simulink model "microduck_nonlinear_state_feedback"  (R2026b)
settings: Solver=ode15s  StopTime=r.test.duration  MaxStep=r.p.cfg.sim.maxStep  RelTol=r.p.cfg.sim.relTol  AbsTol=r.p.cfg.sim.absTol
PreLoadFcn:
  | root=fileparts(get_param(bdroot,'FileName')); addpath(root,fullfile(root,'helpers')); md_expanded_cache;
PostLoadFcn:
  | md_sf_apply(bdroot);
InitFcn:
  | md_sf_apply(bdroot);
model workspace (MAT data in the model file):
  G11 = [-0.6  0; 0  -0.6]
  G12 = -12
  G13 = -4000
  G14 = [-0.6  0; 0  -0.6]
  G15 = -12
  G16 = -4000
  G17 = [-0.6  0; 0  -0.6]
  G18 = -12
  G19 = -4000
  G20 = [-0.6  0; 0  -0.6]
  G21 = -12
  G22 = -4000
  G23 = [-0.6  0; 0  -0.6]
  G24 = -12
  G25 = -4000
  G26 = [-0.6  0; 0  -0.6]
  G27 = -12
  G28 = -4000
  G29 = [-0.6  0; 0  -0.6]
  G30 = -12
  G31 = -4000
  G32 = [-0.6  0; 0  -0.6]
  G33 = -12
  G34 = -4000
  G35 = [0 0 0 0 0 0 1 0 0 0 0 0 ... (112 elements, 14x8)]
  G36 = [0 0 0 0 0 0 0.053 0 0 0 0 0 ... (112 elements, 14x8)]
  G39 = [33.3333333333 0 0 0 0 0 0 0 0 33.3333333333 0 0 ... (64 elements, 8x8)]
  G40 = [0 0 0 0 0 0 0 0 0 0 0 0 ... (112 elements, 8x14)]
  G41 = [0 0 0 0 0 0 0 0 0 0 0 0 ... (112 elements, 8x14)]
  Kd_servo = [0 0 0 0 0 0 0 0 0 0 0 0 ... (64 elements, 8x8)]
  Kp_servo = [0.55 0 0 0 0 0 0 0 0 0.55 0 0 ... (64 elements, 8x8)]
  c10 = 0
  c11 = 0
  c13 = 0
  c14 = 0
  c16 = 0
  c17 = 0
  c19 = 0
  c20 = 0
  c22 = 0
  c23 = 0
  c25 = 0
  c26 = 0
  c4 = 0
  c5 = 0
  c7 = 0
  c8 = 0
  g_world = [0; 0; -9.81]
  push_wrench = [1; 0; 0; 0; 0; 0]
  r : object (value not decoded)
  v_s2 = 2.5e-05
symbols that are objects in the model workspace (value not decoded): r
(part 2 of 5)

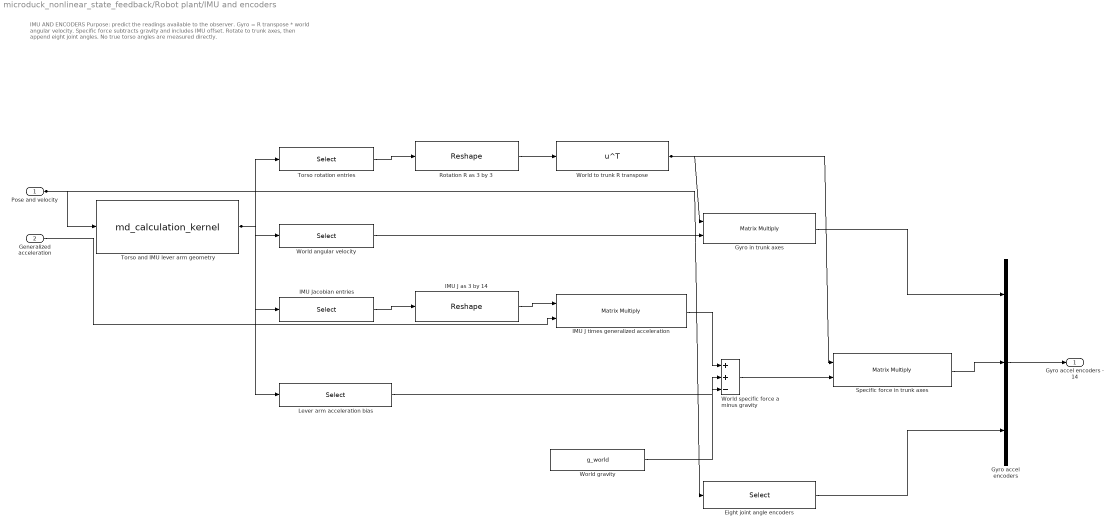
== system microduck_nonlinear_state_feedback/Robot plant/IMU and encoders ==
  note: IMU AND ENCODERS
      |
      | Purpose: predict the readings available to the observer.
      | Gyro = R transpose * world angular velocity. Specific force subtracts gravity and includes IMU offset.
      | Rotate to trunk axes, then append eight joint angles. No true torso angles are measured directly.
  Pose and velocity : Inport  Description=|
      | Pose and velocity
      | 
      | WHAT THIS BLOCK DOES
      | Receives this named signal from the parent folder. Check the name for its meaning and units.
      | 
      | FOLDER CONTEXT
      | IMU AND ENCODERS
      | 
      | Purpose: predict the readings available to the observer.
      | Gyro = R transpose * world angular velocity. Specific force subtracts gravity and includes IMU offset.
      | Rotate to trunk axes, then append eight joint angles. No true torso angles are measured directly.
  Generalized acceleration : Inport  Description=|  Port=2
      | Generalized acceleration
      | 
      | WHAT THIS BLOCK DOES
      | Receives this named signal from the parent folder. Check the name for its meaning and units.
      | 
      | FOLDER CONTEXT
      | IMU AND ENCODERS
      | 
      | Purpose: predict the readings available to the observer.
      | Gyro = R transpose * world angular velocity. Specific force subtracts gravity and includes IMU offset.
      | Rotate to trunk axes, then append eight joint angles. No true torso angles are measured directly.
  Eight joint angle encoders : Selector  Description=|  InputPortWidth=28  IndexOptions=Index vector (dialog)  Indices=[7 8 9 10 11 12 13 14]  OutputSizes=1
      | Eight joint angle encoders
      | 
      | WHAT THIS BLOCK DOES
      | Selects the labelled coordinates from an input vector without changing their physical values. Open the block to see the one-based index list.
      | 
      | FOLDER CONTEXT
      | IMU AND ENCODERS
      | 
      | Purpose: predict the readings available to the observer.
      | Gyro = R transpose * world angular velocity. Specific force subtracts gravity and includes IMU offset.
      | Rotate to trunk axes, then append eight joint angles. No true torso angles are measured directly.
  Gyro accel encoders : Mux  Description=|  Inputs=3
      | Gyro accel encoders
      | 
      | WHAT THIS BLOCK DOES
      | Joins the input vectors in port order, top to bottom. This packages signals; it does not add forces or mix units.
      | 
      | FOLDER CONTEXT
      | IMU AND ENCODERS
      | 
      | Purpose: predict the readings available to the observer.
      | Gyro = R transpose * world angular velocity. Specific force subtracts gravity and includes IMU offset.
      | Rotate to trunk axes, then append eight joint angles. No true torso angles are measured directly.
  Gyro in trunk axes : Product  Description=|  Inputs=**  Multiplication=Matrix(*)
      | Gyro in trunk axes
      | 
      | WHAT THIS BLOCK DOES
      | Multiplies/divides the inputs according to the block settings. Input operations: **. The matrix/vector dimensions must agree.
      | 
      | FOLDER CONTEXT
      | IMU AND ENCODERS
      | 
      | Purpose: predict the readings available to the observer.
      | Gyro = R transpose * world angular velocity. Specific force subtracts gravity and includes IMU offset.
      | Rotate to trunk axes, then append eight joint angles. No true torso angles are measured directly.
  IMU J as 3 by 14 : Reshape  Description=|  OutputDimensionality=Customize  OutputDimensions=[3 14]
      | IMU J as 3 by 14
      | 
      | WHAT THIS BLOCK DOES
      | Changes the arrangement of the entries into the labelled matrix shape. Entries retain MATLAB column-major order and their values do not change.
      | 
      | FOLDER CONTEXT
      | IMU AND ENCODERS
      | 
      | Purpose: predict the readings available to the observer.
      | Gyro = R transpose * world angular velocity. Specific force subtracts gravity and includes IMU offset.
      | Rotate to trunk axes, then append eight joint angles. No true torso angles are measured directly.
  IMU J times generalized acceleration : Product  Description=|  Inputs=**  Multiplication=Matrix(*)
      | IMU J times generalized acceleration
      | 
      | WHAT THIS BLOCK DOES
      | Multiplies/divides the inputs according to the block settings. Input operations: **. The matrix/vector dimensions must agree.
      | 
      | FOLDER CONTEXT
      | IMU AND ENCODERS
      | 
      | Purpose: predict the readings available to the observer.
      | Gyro = R transpose * world angular velocity. Specific force subtracts gravity and includes IMU offset.
      | Rotate to trunk axes, then append eight joint angles. No true torso angles are measured directly.
  IMU Jacobian entries : Selector  Description=|  InputPortWidth=57  IndexOptions=Index vector (dialog)  Indices=[13 14 15 16 17 18 19 20 21 22 23 24 25 26 27 28 29 30 31 32 33 34 35 36 37 38 39 40 41 42 43 44 45 46 47 48 49 50 51 52 53 54]  OutputSizes=1
      | IMU Jacobian entries
      | 
      | WHAT THIS BLOCK DOES
      | Selects the labelled coordinates from an input vector without changing their physical values. Open the block to see the one-based index list.
      | 
      | FOLDER CONTEXT
      | IMU AND ENCODERS
      | 
      | Purpose: predict the readings available to the observer.
      | Gyro = R transpose * world angular velocity. Specific force subtracts gravity and includes IMU offset.
      | Rotate to trunk axes, then append eight joint angles. No true torso angles are measured directly.
  Lever arm acceleration bias : Selector  Description=|  InputPortWidth=57  IndexOptions=Index vector (dialog)  Indices=[55 56 57]  OutputSizes=1
      | Lever arm acceleration bias
      | 
      | WHAT THIS BLOCK DOES
      | Selects the labelled coordinates from an input vector without changing their physical values. Open the block to see the one-based index list.
      | 
      | FOLDER CONTEXT
      | IMU AND ENCODERS
      | 
      | Purpose: predict the readings available to the observer.
      | Gyro = R transpose * world angular velocity. Specific force subtracts gravity and includes IMU offset.
      | Rotate to trunk axes, then append eight joint angles. No true torso angles are measured directly.
  Rotation R as 3 by 3 : Reshape  Description=|  OutputDimensionality=Customize  OutputDimensions=[3 3]
      | Rotation R as 3 by 3
      | 
      | WHAT THIS BLOCK DOES
      | Changes the arrangement of the entries into the labelled matrix shape. Entries retain MATLAB column-major order and their values do not change.
      | 
      | FOLDER CONTEXT
      | IMU AND ENCODERS
      | 
      | Purpose: predict the readings available to the observer.
      | Gyro = R transpose * world angular velocity. Specific force subtracts gravity and includes IMU offset.
      | Rotate to trunk axes, then append eight joint angles. No true torso angles are measured directly.
  Specific force in trunk axes : Product  Description=|  Inputs=**  Multiplication=Matrix(*)
      | Specific force in trunk axes
      | 
      | WHAT THIS BLOCK DOES
      | Multiplies/divides the inputs according to the block settings. Input operations: **. The matrix/vector dimensions must agree.
      | 
      | FOLDER CONTEXT
      | IMU AND ENCODERS
      | 
      | Purpose: predict the readings available to the observer.
      | Gyro = R transpose * world angular velocity. Specific force subtracts gravity and includes IMU offset.
      | Rotate to trunk axes, then append eight joint angles. No true torso angles are measured directly.
  Torso and IMU lever arm geometry : M-S-Function  Description=|  FunctionName=md_calculation_kernel  Parameters=r.p, 'imu_geometry'
      | Torso and IMU lever arm geometry
      | 
      | WHAT THIS BLOCK DOES
      | Performs the mathematical operation named on this block. Open its parameter dialog to inspect the operator and dimensions.
      | 
      | FOLDER CONTEXT
      | IMU AND ENCODERS
      | 
      | Purpose: predict the readings available to the observer.
      | Gyro = R transpose * world angular velocity. Specific force subtracts gravity and includes IMU offset.
      | Rotate to trunk axes, then append eight joint angles. No true torso angles are measured directly.
      settings: OpenFcn=edit md_rigid_body_math; edit md_calculation_kernel;
  Torso rotation entries : Selector  Description=|  InputPortWidth=57  IndexOptions=Index vector (dialog)  Indices=[1 2 3 4 5 6 7 8 9]  OutputSizes=1
      | Torso rotation entries
      | 
      | WHAT THIS BLOCK DOES
      | Selects the labelled coordinates from an input vector without changing their physical values. Open the block to see the one-based index list.
      | 
      | FOLDER CONTEXT
      | IMU AND ENCODERS
      | 
      | Purpose: predict the readings available to the observer.
      | Gyro = R transpose * world angular velocity. Specific force subtracts gravity and includes IMU offset.
      | Rotate to trunk axes, then append eight joint angles. No true torso angles are measured directly.
  World angular velocity : Selector  Description=|  InputPortWidth=57  IndexOptions=Index vector (dialog)  Indices=[10 11 12]  OutputSizes=1
      | World angular velocity
      | 
      | WHAT THIS BLOCK DOES
      | Selects the labelled coordinates from an input vector without changing their physical values. Open the block to see the one-based index list.
      | 
      | FOLDER CONTEXT
      | IMU AND ENCODERS
      | 
      | Purpose: predict the readings available to the observer.
      | Gyro = R transpose * world angular velocity. Specific force subtracts gravity and includes IMU offset.
      | Rotate to trunk axes, then append eight joint angles. No true torso angles are measured directly.
  World gravity : Constant  Description=|  Value=g_world
      | SHARED PARAMETER: g_world = r.p.g
      | Edit sf_parameters.m; per-model edits are refreshed on Run.
      | 
      | WHAT THIS BLOCK DOES
      | World gravity
      | 
      | PARAMETER
      | g_world = r.p.g
      | 
      | The short symbol is stored in this model workspace. Its numeric value is unchanged from the validated model.
  World specific force a minus gravity : Sum  Description=|  Inputs=++-
      | World specific force a minus gravity
      | 
      | WHAT THIS BLOCK DOES
      | Combines its inputs using the plus/minus signs shown on the icon. Signs: ++-.
      | 
      | FOLDER CONTEXT
      | IMU AND ENCODERS
      | 
      | Purpose: predict the readings available to the observer.
      | Gyro = R transpose * world angular velocity. Specific force subtracts gravity and includes IMU offset.
      | Rotate to trunk axes, then append eight joint angles. No true torso angles are measured directly.
  World to trunk R transpose : Math  Description=|  Operator=transpose
      | World to trunk R transpose
      | 
      | WHAT THIS BLOCK DOES
      | Performs the mathematical operation named on this block. Open its parameter dialog to inspect the operator and dimensions.
      | 
      | FOLDER CONTEXT
      | IMU AND ENCODERS
      | 
      | Purpose: predict the readings available to the observer.
      | Gyro = R transpose * world angular velocity. Specific force subtracts gravity and includes IMU offset.
      | Rotate to trunk axes, then append eight joint angles. No true torso angles are measured directly.
  Gyro accel encoders - 14 : Outport  Description=|
      | Gyro accel encoders - 14
      | 
      | WHAT THIS BLOCK DOES
      | Carries this named result out of the folder. The port number defines the interface order.
      | 
      | FOLDER CONTEXT
      | IMU AND ENCODERS
      | 
      | Purpose: predict the readings available to the observer.
      | Gyro = R transpose * world angular velocity. Specific force subtracts gravity and includes IMU offset.
      | Rotate to trunk axes, then append eight joint angles. No true torso angles are measured directly.
  wires:
  Pose and velocity/1 -> Eight joint angle encoders/1, Torso and IMU lever arm geometry/1
  Gyro in trunk axes/1 -> Gyro accel encoders/1
  Specific force in trunk axes/1 -> Gyro accel encoders/2
  Eight joint angle encoders/1 -> Gyro accel encoders/3
  World to trunk R transpose/1 -> Gyro in trunk axes/1, Specific force in trunk axes/1
  World angular velocity/1 -> Gyro in trunk axes/2
  IMU Jacobian entries/1 -> IMU J as 3 by 14/1
  IMU J as 3 by 14/1 -> IMU J times generalized acceleration/1
  Generalized acceleration/1 -> IMU J times generalized acceleration/2
  Torso and IMU lever arm geometry/1 -> IMU Jacobian entries/1, Lever arm acceleration bias/1, Torso rotation entries/1, World angular velocity/1
  Torso rotation entries/1 -> Rotation R as 3 by 3/1
  World specific force a minus gravity/1 -> Specific force in trunk axes/2
  IMU J times generalized acceleration/1 -> World specific force a minus gravity/1
  Lever arm acceleration bias/1 -> World specific force a minus gravity/2
  World gravity/1 -> World specific force a minus gravity/3
  Rotation R as 3 by 3/1 -> World to trunk R transpose/1
  Gyro accel encoders/1 -> Gyro accel encoders - 14/1

== system microduck_nonlinear_state_feedback/Robot plant/Integrate body motion ==
  note: INTEGRATE BODY MOTION
      |
      | Purpose: convert generalized acceleration into the robot pose over time.
      | First integrator: acceleration -> velocity v. Second integrator: velocity -> coordinates q.
      | The initial pose is the trimmed standing equilibrium. q and v each contain 14 values.
  In1 : Inport  Description=|
      | In1
      | 
      | WHAT THIS BLOCK DOES
      | Receives this named signal from the parent folder. Check the name for its meaning and units.
      | 
      | FOLDER CONTEXT
      | INTEGRATE BODY MOTION
      | 
      | Purpose: convert generalized acceleration into the robot pose over time.
      | First integrator: acceleration -> velocity v. Second integrator: velocity -> coordinates q.
      | The initial pose is the trimmed standing equilibrium. q and v each contain 14 values.
  Generalized velocities v : Integrator  Description=|  InitialCondition=zeros(14,1)
      | Generalized velocities v
      | 
      | WHAT THIS BLOCK DOES
      | Continuous state memory: integrates the input over time. Starts at InitialCondition = zeros(14,1).
      | 
      | FOLDER CONTEXT
      | INTEGRATE BODY MOTION
      | 
      | Purpose: convert generalized acceleration into the robot pose over time.
      | First integrator: acceleration -> velocity v. Second integrator: velocity -> coordinates q.
      | The initial pose is the trimmed standing equilibrium. q and v each contain 14 values.
  Joint and body coordinates q : Integrator  Description=|  InitialCondition=r.p.xeq(1:14)
      | Joint and body coordinates q
      | 
      | WHAT THIS BLOCK DOES
      | Continuous state memory: integrates the input over time. Starts at InitialCondition = r.p.xeq(1:14).
      | 
      | FOLDER CONTEXT
      | INTEGRATE BODY MOTION
      | 
      | Purpose: convert generalized acceleration into the robot pose over time.
      | First integrator: acceleration -> velocity v. Second integrator: velocity -> coordinates q.
      | The initial pose is the trimmed standing equilibrium. q and v each contain 14 values.
  q and v : Mux  Description=|  Inputs=2
      | q and v
      | 
      | WHAT THIS BLOCK DOES
      | Joins the input vectors in port order, top to bottom. This packages signals; it does not add forces or mix units.
      | 
      | FOLDER CONTEXT
      | INTEGRATE BODY MOTION
      | 
      | Purpose: convert generalized acceleration into the robot pose over time.
      | First integrator: acceleration -> velocity v. Second integrator: velocity -> coordinates q.
      | The initial pose is the trimmed standing equilibrium. q and v each contain 14 values.
  Out1 : Outport  Description=|
      | Out1
      | 
      | WHAT THIS BLOCK DOES
      | Carries this named result out of the folder. The port number defines the interface order.
      | 
      | FOLDER CONTEXT
      | INTEGRATE BODY MOTION
      | 
      | Purpose: convert generalized acceleration into the robot pose over time.
      | First integrator: acceleration -> velocity v. Second integrator: velocity -> coordinates q.
      | The initial pose is the trimmed standing equilibrium. q and v each contain 14 values.
  Out2 : Outport  Description=|  Port=2
      | Out2
      | 
      | WHAT THIS BLOCK DOES
      | Carries this named result out of the folder. The port number defines the interface order.
      | 
      | FOLDER CONTEXT
      | INTEGRATE BODY MOTION
      | 
      | Purpose: convert generalized acceleration into the robot pose over time.
      | First integrator: acceleration -> velocity v. Second integrator: velocity -> coordinates q.
      | The initial pose is the trimmed standing equilibrium. q and v each contain 14 values.
  Out3 : Outport  Description=|  Port=3
      | Out3
      | 
      | WHAT THIS BLOCK DOES
      | Carries this named result out of the folder. The port number defines the interface order.
      | 
      | FOLDER CONTEXT
      | INTEGRATE BODY MOTION
      | 
      | Purpose: convert generalized acceleration into the robot pose over time.
      | First integrator: acceleration -> velocity v. Second integrator: velocity -> coordinates q.
      | The initial pose is the trimmed standing equilibrium. q and v each contain 14 values.
  wires:
  In1/1 -> Generalized velocities v/1
  Generalized velocities v/1 -> Joint and body coordinates q/1, q and v/2, Out3/1
  Joint and body coordinates q/1 -> q and v/1, Out1/1
  q and v/1 -> Out2/1

== system microduck_nonlinear_state_feedback/Robot plant/Rigid body force balance ==
  note: RIGID BODY FORCE BALANCE
      |
      | Purpose: combine all physical forces and solve for acceleration.
      | M * acceleration = motor + contact + push - gravity and velocity bias - damping.
      | M couples the body and joints, so acceleration is found with one matrix solve.
  Pose and velocity : Inport  Description=|
      | Pose and velocity
      | 
      | WHAT THIS BLOCK DOES
      | Receives this named signal from the parent folder. Check the name for its meaning and units.
      | 
      | FOLDER CONTEXT
      | RIGID BODY FORCE BALANCE
      | 
      | Purpose: combine all physical forces and solve for acceleration.
      | M * acceleration = motor + contact + push - gravity and velocity bias - damping.
      | M couples the body and joints, so acceleration is found with one matrix solve.
  Motor torques : Inport  Description=|  Port=2
      | Motor torques
      | 
      | WHAT THIS BLOCK DOES
      | Receives this named signal from the parent folder. Check the name for its meaning and units.
      | 
      | FOLDER CONTEXT
      | RIGID BODY FORCE BALANCE
      | 
      | Purpose: combine all physical forces and solve for acceleration.
      | M * acceleration = motor + contact + push - gravity and velocity bias - damping.
      | M couples the body and joints, so acceleration is found with one matrix solve.
  Ground forces : Inport  Description=|  Port=3
      | Ground forces
      | 
      | WHAT THIS BLOCK DOES
      | Receives this named signal from the parent folder. Check the name for its meaning and units.
      | 
      | FOLDER CONTEXT
      | RIGID BODY FORCE BALANCE
      | 
      | Purpose: combine all physical forces and solve for acceleration.
      | M * acceleration = motor + contact + push - gravity and velocity bias - damping.
      | M couples the body and joints, so acceleration is found with one matrix solve.
  External wrench : Inport  Description=|  Port=4
      | External wrench
      | 
      | WHAT THIS BLOCK DOES
      | Receives this named signal from the parent folder. Check the name for its meaning and units.
      | 
      | FOLDER CONTEXT
      | RIGID BODY FORCE BALANCE
      | 
      | Purpose: combine all physical forces and solve for acceleration.
      | M * acceleration = motor + contact + push - gravity and velocity bias - damping.
      | M couples the body and joints, so acceleration is found with one matrix solve.
  Apply eight motor torques : Gain  Description=|  Gain=G35  Multiplication=Matrix(K*u)
      | SHARED PARAMETER: G35 = r.p.S
      | Edit sf_parameters.m; per-model edits are refreshed on Run.
      | 
      | WHAT THIS BLOCK DOES
      | Apply eight motor torques
      | 
      | PARAMETER
      | G35 = r.p.S
      | 
      | The short symbol is stored in this model workspace. Its numeric value is unchanged from the validated model.
  Bias h gravity and inertial : Selector  Description=|  InputPortWidth=210  IndexOptions=Index vector (dialog)  Indices=[197 198 199 200 201 202 203 204 205 206 207 208 209 210]  OutputSizes=1
      | Bias h gravity and inertial
      | 
      | WHAT THIS BLOCK DOES
      | Selects the labelled coordinates from an input vector without changing their physical values. Open the block to see the one-based index list.
      | 
      | FOLDER CONTEXT
      | RIGID BODY FORCE BALANCE
      | 
      | Purpose: combine all physical forces and solve for acceleration.
      | M * acceleration = motor + contact + push - gravity and velocity bias - damping.
      | M couples the body and joints, so acceleration is found with one matrix solve.
  Joint velocities : Selector  Description=|  InputPortWidth=28  IndexOptions=Index vector (dialog)  Indices=[21 22 23 24 25 26 27 28]  OutputSizes=1
      | Joint velocities
      | 
      | WHAT THIS BLOCK DOES
      | Selects the labelled coordinates from an input vector without changing their physical values. Open the block to see the one-based index list.
      | 
      | FOLDER CONTEXT
      | RIGID BODY FORCE BALANCE
      | 
      | Purpose: combine all physical forces and solve for acceleration.
      | M * acceleration = motor + contact + push - gravity and velocity bias - damping.
      | M couples the body and joints, so acceleration is found with one matrix solve.
  M as 14 by 14 : Reshape  Description=|  OutputDimensionality=Customize  OutputDimensions=[14 14]
      | M as 14 by 14
      | 
      | WHAT THIS BLOCK DOES
      | Changes the arrangement of the entries into the labelled matrix shape. Entries retain MATLAB column-major order and their values do not change.
      | 
      | FOLDER CONTEXT
      | RIGID BODY FORCE BALANCE
      | 
      | Purpose: combine all physical forces and solve for acceleration.
      | M * acceleration = motor + contact + push - gravity and velocity bias - damping.
      | M couples the body and joints, so acceleration is found with one matrix solve.
  Mass matrix and gravity velocity bias : M-S-Function  Description=|  FunctionName=md_calculation_kernel  Parameters=r.p, 'mass'
      | Mass matrix and gravity velocity bias
      | 
      | WHAT THIS BLOCK DOES
      | Performs the mathematical operation named on this block. Open its parameter dialog to inspect the operator and dimensions.
      | 
      | FOLDER CONTEXT
      | RIGID BODY FORCE BALANCE
      | 
      | Purpose: combine all physical forces and solve for acceleration.
      | M * acceleration = motor + contact + push - gravity and velocity bias - damping.
      | M couples the body and joints, so acceleration is found with one matrix solve.
      settings: OpenFcn=edit md_rigid_body_math; edit md_calculation_kernel;
  Mass matrix entries : Selector  Description=|  InputPortWidth=210  IndexOptions=Index vector (dialog)  Indices=[1 2 3 4 5 6 7 8 9 10 11 12 13 14 15 16 17 18 19 20 21 22 23 24 25 26 27 28 29 30 31 32 33 34 35 36 37 38 39 40 41 42 43 44 45 46 47 48 49 50 51 52 53 54 55 56 57 58 59 60 61 62 63 64 65 66 67 68 69 70 71 72 73 74 75 76 77 78 79 80 81 82 83 84 85 86 87 88 89 90 91 92 93 94 95 96 97 98 99 100 101 102 103 104 105 106 107 108 109 110 111 112 113 114 115 116 117 118 119 120 121 122 123 124 125 126 127 128 129 130 131 132 133 134 135 136 137 138 139 140 141 142 143 144 145 146 147 148 149 150 151 152 153 154 155 156 157 158 159 160 161 162 163 164 165 166 167 168 169 170 171 172 173 174 175 176 177 178 179 180 181 182 183 184 185 186 187 188 189 190 191 192 193 194 195 196]  OutputSizes=1
      | Mass matrix entries
      | 
      | WHAT THIS BLOCK DOES
      | Selects the labelled coordinates from an input vector without changing their physical values. Open the block to see the one-based index list.
      | 
      | FOLDER CONTEXT
      | RIGID BODY FORCE BALANCE
      | 
      | Purpose: combine all physical forces and solve for acceleration.
      | M * acceleration = motor + contact + push - gravity and velocity bias - damping.
      | M couples the body and joints, so acceleration is found with one matrix solve.
  Mechanical joint damping : Gain  Description=|  Gain=G36  Multiplication=Matrix(K*u)
      | SHARED PARAMETER: G36 = [zeros(6,8);diag(r.p.bjoint)]
      | Edit sf_parameters.m; per-model edits are refreshed on Run.
      | 
      | WHAT THIS BLOCK DOES
      | Mechanical joint damping
      | 
      | PARAMETER
      | G36 = [zeros(6,8);diag(r.p.bjoint)]
      | 
      | The short symbol is stored in this model workspace. Its numeric value is unchanged from the validated model.
  Net generalized force : Sum  Description=|  Inputs=+++--
      | Net generalized force
      | 
      | WHAT THIS BLOCK DOES
      | Combines its inputs using the plus/minus signs shown on the icon. Signs: +++--.
      | 
      | FOLDER CONTEXT
      | RIGID BODY FORCE BALANCE
      | 
      | Purpose: combine all physical forces and solve for acceleration.
      | M * acceleration = motor + contact + push - gravity and velocity bias - damping.
      | M couples the body and joints, so acceleration is found with one matrix solve.
  Pose velocity and world wrench : Mux  Description=|  Inputs=2
      | Pose velocity and world wrench
      | 
      | WHAT THIS BLOCK DOES
      | Joins the input vectors in port order, top to bottom. This packages signals; it does not add forces or mix units.
      | 
      | FOLDER CONTEXT
      | RIGID BODY FORCE BALANCE
      | 
      | Purpose: combine all physical forces and solve for acceleration.
      | M * acceleration = motor + contact + push - gravity and velocity bias - damping.
      | M couples the body and joints, so acceleration is found with one matrix solve.
  Project torso wrench with Jacobians : M-S-Function  Description=|  FunctionName=md_calculation_kernel  Parameters=r.p, 'wrench'
      | Project torso wrench with Jacobians
      | 
      | WHAT THIS BLOCK DOES
      | Performs the mathematical operation named on this block. Open its parameter dialog to inspect the operator and dimensions.
      | 
      | FOLDER CONTEXT
      | RIGID BODY FORCE BALANCE
      | 
      | Purpose: combine all physical forces and solve for acceleration.
      | M * acceleration = motor + contact + push - gravity and velocity bias - damping.
      | M couples the body and joints, so acceleration is found with one matrix solve.
      settings: OpenFcn=edit md_rigid_body_math; edit md_calculation_kernel;
  Solve M times acceleration equals force : MATLAB Function  Description=|  TreatAsAtomicUnit=on
      | RIGID BODY FORCE BALANCE
      | 
      | Purpose: combine all physical forces and solve for acceleration.
      | M * acceleration = motor + contact + push - gravity and velocity bias - damping.
      | M couples the body and joints, so acceleration is found with one matrix solve.
  Acceleration - 14 : Outport  Description=|
      | Acceleration - 14
      | 
      | WHAT THIS BLOCK DOES
      | Carries this named result out of the folder. The port number defines the interface order.
      | 
      | FOLDER CONTEXT
      | RIGID BODY FORCE BALANCE
      | 
      | Purpose: combine all physical forces and solve for acceleration.
      | M * acceleration = motor + contact + push - gravity and velocity bias - damping.
      | M couples the body and joints, so acceleration is found with one matrix solve.
  wires:
  Motor torques/1 -> Apply eight motor torques/1
  Mass matrix and gravity velocity bias/1 -> Bias h gravity and inertial/1, Mass matrix entries/1
  Pose and velocity/1 -> Joint velocities/1, Mass matrix and gravity velocity bias/1, Pose velocity and world wrench/1
  Mass matrix entries/1 -> M as 14 by 14/1
  Joint velocities/1 -> Mechanical joint damping/1
  Apply eight motor torques/1 -> Net generalized force/1
  Ground forces/1 -> Net generalized force/2
  Project torso wrench with Jacobians/1 -> Net generalized force/3
  Bias h gravity and inertial/1 -> Net generalized force/4
  Mechanical joint damping/1 -> Net generalized force/5
  External wrench/1 -> Pose velocity and world wrench/2
  Pose velocity and world wrench/1 -> Project torso wrench with Jacobians/1
  M as 14 by 14/1 -> Solve M times acceleration equals force/1(M)
  Net generalized force/1 -> Solve M times acceleration equals force/2(force)
  Solve M times acceleration equals force/1(acceleration) -> Acceleration - 14/1

== system microduck_nonlinear_state_feedback/Robot plant/Servo position control ==
  note: SERVO POSITION CONTROL
      |
      | Purpose: model the eight internal position servos, including their response delay.
      | Angle error -> internal PD torque -> torque limit -> first-order torque lag.
      | These inner loops are part of the plant; the outer balance PID changes their targets.
  Desired angles u : Inport  Description=|
      | Desired angles u
      | 
      | WHAT THIS BLOCK DOES
      | Receives this named signal from the parent folder. Check the name for its meaning and units.
      | 
      | FOLDER CONTEXT
      | SERVO POSITION CONTROL
      | 
      | Purpose: model the eight internal position servos, including their response delay.
      | Angle error -> internal PD torque -> torque limit -> first-order torque lag.
      | These inner loops are part of the plant; the outer balance PID changes their targets.
  Coordinates q : Inport  Description=|  Port=2
      | Coordinates q
      | 
      | WHAT THIS BLOCK DOES
      | Receives this named signal from the parent folder. Check the name for its meaning and units.
      | 
      | FOLDER CONTEXT
      | SERVO POSITION CONTROL
      | 
      | Purpose: model the eight internal position servos, including their response delay.
      | Angle error -> internal PD torque -> torque limit -> first-order torque lag.
      | These inner loops are part of the plant; the outer balance PID changes their targets.
  Velocities v : Inport  Description=|  Port=3
      | Velocities v
      | 
      | WHAT THIS BLOCK DOES
      | Receives this named signal from the parent folder. Check the name for its meaning and units.
      | 
      | FOLDER CONTEXT
      | SERVO POSITION CONTROL
      | 
      | Purpose: model the eight internal position servos, including their response delay.
      | Angle error -> internal PD torque -> torque limit -> first-order torque lag.
      | These inner loops are part of the plant; the outer balance PID changes their targets.
  Actual motor torques : Integrator  Description=|  InitialCondition=r.p.xeq(29:36)
      | Actual motor torques
      | 
      | WHAT THIS BLOCK DOES
      | Continuous state memory: integrates the input over time. Starts at InitialCondition = r.p.xeq(29:36).
      | 
      | FOLDER CONTEXT
      | SERVO POSITION CONTROL
      | 
      | Purpose: model the eight internal position servos, including their response delay.
      | Angle error -> internal PD torque -> torque limit -> first-order torque lag.
      | These inner loops are part of the plant; the outer balance PID changes their targets.
  Desired angle limits : Saturate  Description=|  UpperLimit=r.p.jointMax  LowerLimit=r.p.jointMin
      | Desired angle limits
      | 
      | WHAT THIS BLOCK DOES
      | Clips each input element to the permitted interval. Lower bound: r.p.jointMin. Upper bound: r.p.jointMax.
      | 
      | FOLDER CONTEXT
      | SERVO POSITION CONTROL
      | 
      | Purpose: model the eight internal position servos, including their response delay.
      | Angle error -> internal PD torque -> torque limit -> first-order torque lag.
      | These inner loops are part of the plant; the outer balance PID changes their targets.
  Internal derivative gain : Gain  Description=|  Gain=Kd_servo  Multiplication=Matrix(K*u)
      | SHARED PARAMETER: Kd_servo = diag(r.p.kd)
      | Edit sf_parameters.m; per-model edits are refreshed on Run.
      | 
      | WHAT THIS BLOCK DOES
      | Internal derivative gain
      | 
      | PARAMETER
      | Kd_servo = diag(r.p.kd)
      | 
      | The short symbol is stored in this model workspace. Its numeric value is unchanged from the validated model.
  Internal proportional gain : Gain  Description=|  Gain=Kp_servo  Multiplication=Matrix(K*u)
      | SHARED PARAMETER: Kp_servo = diag(r.p.kp)
      | Edit sf_parameters.m; per-model edits are refreshed on Run.
      | 
      | WHAT THIS BLOCK DOES
      | Internal proportional gain
      | 
      | PARAMETER
      | Kp_servo = diag(r.p.kp)
      | 
      | The short symbol is stored in this model workspace. Its numeric value is unchanged from the validated model.
  Inverse servo time constant : Gain  Description=|  Gain=G39  Multiplication=Matrix(K*u)
      | SHARED PARAMETER: G39 = diag(1./r.p.Ta)
      | Edit sf_parameters.m; per-model edits are refreshed on Run.
      | 
      | WHAT THIS BLOCK DOES
      | Inverse servo time constant
      | 
      | PARAMETER
      | G39 = diag(1./r.p.Ta)
      | 
      | The short symbol is stored in this model workspace. Its numeric value is unchanged from the validated model.
  Motor target torque limits : Saturate  Description=|  UpperLimit=r.p.tauMax  LowerLimit=-r.p.tauMax
      | Motor target torque limits
      | 
      | WHAT THIS BLOCK DOES
      | Clips each input element to the permitted interval. Lower bound: -r.p.tauMax. Upper bound: r.p.tauMax.
      | 
      | FOLDER CONTEXT
      | SERVO POSITION CONTROL
      | 
      | Purpose: model the eight internal position servos, including their response delay.
      | Angle error -> internal PD torque -> torque limit -> first-order torque lag.
      | These inner loops are part of the plant; the outer balance PID changes their targets.
  Select eight joint angles : Gain  Description=|  Gain=G40  Multiplication=Matrix(K*u)
      | SHARED PARAMETER: G40 = [zeros(8,6) eye(8)]
      | Edit sf_parameters.m; per-model edits are refreshed on Run.
      | 
      | WHAT THIS BLOCK DOES
      | Select eight joint angles
      | 
      | PARAMETER
      | G40 = [zeros(8,6) eye(8)]
      | 
      | The short symbol is stored in this model workspace. Its numeric value is unchanged from the validated model.
  Select eight joint rates : Gain  Description=|  Gain=G41  Multiplication=Matrix(K*u)
      | SHARED PARAMETER: G41 = [zeros(8,6) eye(8)]
      | Edit sf_parameters.m; per-model edits are refreshed on Run.
      | 
      | WHAT THIS BLOCK DOES
      | Select eight joint rates
      | 
      | PARAMETER
      | G41 = [zeros(8,6) eye(8)]
      | 
      | The short symbol is stored in this model workspace. Its numeric value is unchanged from the validated model.
  Servo position error : Sum  Description=|  Inputs=+-
      | Servo position error
      | 
      | WHAT THIS BLOCK DOES
      | Combines its inputs using the plus/minus signs shown on the icon. Signs: +-.
      | 
      | FOLDER CONTEXT
      | SERVO POSITION CONTROL
      | 
      | Purpose: model the eight internal position servos, including their response delay.
      | Angle error -> internal PD torque -> torque limit -> first-order torque lag.
      | These inner loops are part of the plant; the outer balance PID changes their targets.
  Target minus actual torque : Sum  Description=|  Inputs=+-
      | Target minus actual torque
      | 
      | WHAT THIS BLOCK DOES
      | Combines its inputs using the plus/minus signs shown on the icon. Signs: +-.
      | 
      | FOLDER CONTEXT
      | SERVO POSITION CONTROL
      | 
      | Purpose: model the eight internal position servos, including their response delay.
      | Angle error -> internal PD torque -> torque limit -> first-order torque lag.
      | These inner loops are part of the plant; the outer balance PID changes their targets.
  Target torque PD : Sum  Description=|  Inputs=+-
      | Target torque PD
      | 
      | WHAT THIS BLOCK DOES
      | Combines its inputs using the plus/minus signs shown on the icon. Signs: +-.
      | 
      | FOLDER CONTEXT
      | SERVO POSITION CONTROL
      | 
      | Purpose: model the eight internal position servos, including their response delay.
      | Angle error -> internal PD torque -> torque limit -> first-order torque lag.
      | These inner loops are part of the plant; the outer balance PID changes their targets.
  Actual torques tau - Nm : Outport  Description=|
      | Actual torques tau - Nm
      | 
      | WHAT THIS BLOCK DOES
      | Carries this named result out of the folder. The port number defines the interface order.
      | 
      | FOLDER CONTEXT
      | SERVO POSITION CONTROL
      | 
      | Purpose: model the eight internal position servos, including their response delay.
      | Angle error -> internal PD torque -> torque limit -> first-order torque lag.
      | These inner loops are part of the plant; the outer balance PID changes their targets.
  wires:
  Inverse servo time constant/1 -> Actual motor torques/1
  Desired angles u/1 -> Desired angle limits/1
  Select eight joint rates/1 -> Internal derivative gain/1
  Servo position error/1 -> Internal proportional gain/1
  Target minus actual torque/1 -> Inverse servo time constant/1
  Target torque PD/1 -> Motor target torque limits/1
  Coordinates q/1 -> Select eight joint angles/1
  Velocities v/1 -> Select eight joint rates/1
  Desired angle limits/1 -> Servo position error/1
  Select eight joint angles/1 -> Servo position error/2
  Motor target torque limits/1 -> Target minus actual torque/1
  Actual motor torques/1 -> Target minus actual torque/2, Actual torques tau - Nm/1
  Internal proportional gain/1 -> Target torque PD/1
  Internal derivative gain/1 -> Target torque PD/2
